simulink model "RCAM_PID_takeoff_lamding_20261013_step02"  (R2024b)
settings: Solver=VariableStepAuto  StartTime=0.0  StopTime=4200  MaxStep=0.01  RelTol=1e-3
undefined symbols (not defined in the file or in its folder): RCAM_dynamics_fcn20261013_step02_brake, RCAM_monitor_20261013_step02
libraries: simulink x28, slpidlib x9, simulink_extras x2
(part 1 of 2)
settings Model: Creator=rukky  LastModifiedBy=rukky
settings SolverCC: ZeroCrossAlgorithm=Adaptive
settings DebuggingCC: MaskedZcDiagnostic=none  IgnoredZcDiagnostic=none

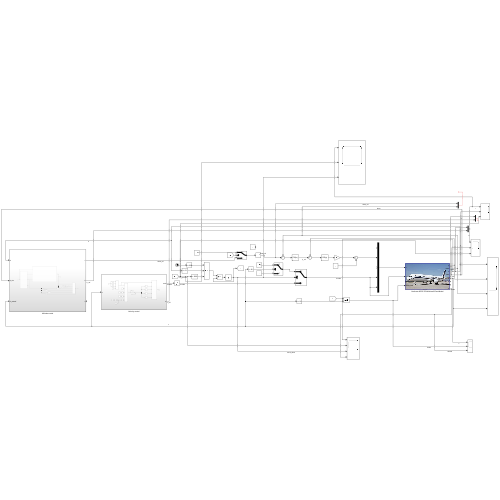
[thumbnail: Simulink's stored preview of the top-level diagram]
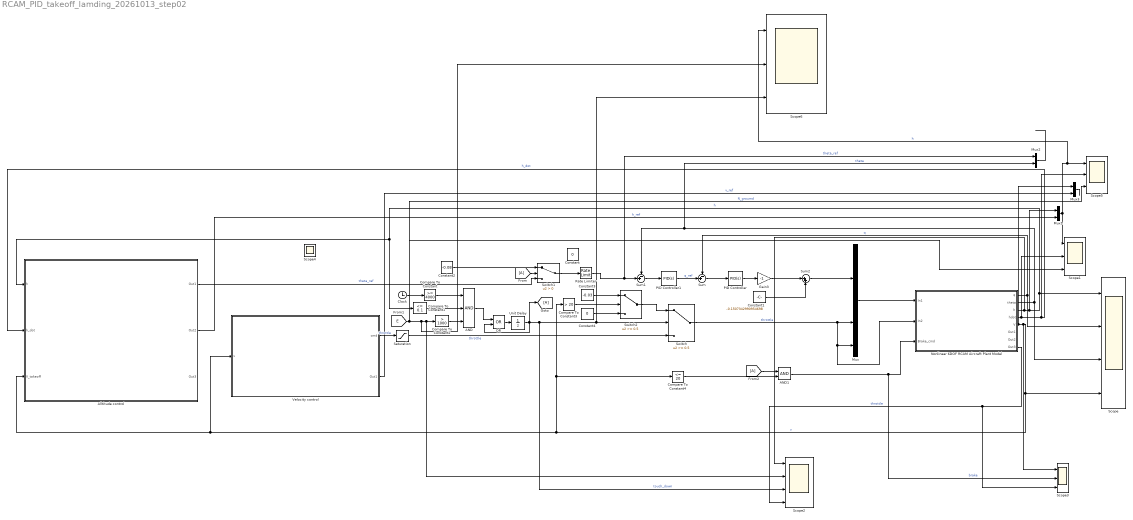
== system RCAM_PID_takeoff_lamding_20261013_step02 ==
  AND : Logic  Inputs=3  AllPortsSameDT=off  OutDataTypeStr=boolean
  AND1 : Logic  AllPortsSameDT=off  OutDataTypeStr=boolean
  Alltitude control : Subsystem
  Clock : Clock
  Compare To Constant : simulink/Logic and Bit Operations/Compare To Constant  relop=>=  const=4000  OutDataTypeStr=boolean
  Compare To Constant1 : simulink/Logic and Bit Operations/Compare To Constant  relop=<=  const=0.1  OutDataTypeStr=boolean
  Compare To Constant2 : simulink/Logic and Bit Operations/Compare To Constant  relop=>  const=1000  OutDataTypeStr=boolean
  Compare To Constant3 : simulink/Logic and Bit Operations/Compare To Constant  relop=>  const=20  OutDataTypeStr=boolean
  Compare To Constant4 : simulink/Logic and Bit Operations/Compare To Constant  relop=<=  const=20  OutDataTypeStr=boolean
  Constant : Constant  Value=0
  Constant1 : Constant  Value=-0.1507342990954698
  Constant2 : Constant  Value=-0.08
  Constant3 : Constant  Value=-0.03
  Constant4 : Constant  Value=0
  From : From
  From2 : From
  Gain3 : Gain  Gain=-1
  Goto : Goto
  Mux : Mux  Inputs=5
  Mux1 : Mux  Inputs=2
  Mux2 : Mux  Inputs=2
  Mux3 : Mux  Inputs=2
  Nonlinear 6DOF RCAM Aircraft Plant Model : Subsystem
      mask Display: image('$imagefile'); % Use "Edit Image" on toolstrip to change.
  OR : Logic  Operator=OR  AllPortsSameDT=off  OutDataTypeStr=boolean
  PID Controller : slpidlib/PID Controller  Controller=PID  Form=Parallel  TimeDomain=Continuous-time  UseExternalTs=off  SampleTime=-1  IntegratorMethod=Forward Euler  FilterMethod=Forward Euler  ControllerParametersSource=internal  P=20  I=20  UseKiTs=off  D=0  UseExternalDerivativeSource=off  N=100  UseFilter=on  TunerSelectOption=Transfer Function Based (PID Tuner App)  InitialConditionSource=internal  InitialConditionForIntegrator=0  InitialConditionForFilter=0  DifferentiatorICPrevScaledInput=0  ExternalReset=none  TrackingMode=off  Kt=1  LimitOutput=off  SatLimitsSource=internal  UpperSaturationLimit=inf  LowerSaturationLimit=-inf  LinearizeAsGain=on  AntiWindupMode=none  Kb=1  LimitIntegrator=off  UpperIntegratorSaturationLimit=inf  LowerIntegratorSaturationLimit=-inf  POutMin=[]  POutMax=[]  IOutMin=[]  IOutMax=[]  DOutMin=[]  DOutMax=[]  NOutMin=[]  NOutMax=[]  SumOutMin=[]  SumOutMax=[]  SaturationOutMin=[]  SaturationOutMax=[]  PParamMin=[]  PParamMax=[]  IParamMin=[]  IParamMax=[]  DParamMin=[]  DParamMax=[]  NParamMin=[]  NParamMax=[]  KbParamMin=[]  KbParamMax=[]  KtParamMin=[]  KtParamMax=[]  KbOutMin=[]  KbOutMax=[]  KtOutMin=[]  KtOutMax=[]  IntegratorOutMin=[]  IntegratorOutMax=[]  FilterOutMin=[]  FilterOutMax=[]  SumI1OutMin=[]  SumI1OutMax=[]  SumI2OutMin=[]  SumI2OutMax=[]  SumI3OutMin=[]  SumI3OutMax=[]  SumI4OutMin=[]  SumI4OutMax=[]  SumDOutMin=[]  SumDOutMax=[]  DifferentiatorOutMin=[]  DifferentiatorOutMax=[]  FilterDiffOutCoefMin=[]  FilterDiffOutCoefMax=[]  ReciprocalOutMin=[]  ReciprocalOutMax=[]  SumDenOutMin=[]  SumDenOutMax=[]  SumNumOutMin=[]  SumNumOutMax=[]  DivideOutMin=[]  DivideOutMax=[]  UdiffTsProdOutMin=[]  UdiffTsProdOutMax=[]  NTsProdOutMin=[]  NTsProdOutMax=[]  UintegralTsProdOutMin=[]  UintegralTsProdOutMax=[]  UngainTsProdOutMin=[]  UngainTsProdOutMax=[]  ClampingZeroOutDataTypeStr=Inherit: Inherit via back propagation  ClampingZeroOutMin=[]  ClampingZeroOutMax=[]  FilterDenConstantOutDataTypeStr=Inherit: Inherit via back propagation  FilterDenConstantOutMin=[]  FilterDenConstantOutMax=[]  PCopyOutDataTypeStr=Inherit: Inherit via back propagation  PCopyOutMin=[]  PCopyOutMax=[]  NCopyOutDataTypeStr=Inherit: Inherit via back propagation  NCopyOutMin=[]  NCopyOutMax=[]  IntegratorContinuousStateAttributes=''  IntegratorStateMustResolveToSignalObject=off  IntegratorRTWStateStorageClass=Auto  FilterContinuousStateAttributes=''  FilterStateMustResolveToSignalObject=off  FilterRTWStateStorageClass=Auto  ParallelPVariant=InternalParameters  IdealPVariant=Disabled  IVariant=InternalParameters  DVariant=InternalParameters  IntegratorVariant=Continuous  SatVariant=Disabled  AWVariant=Passthrough  PCopyVariant=Disabled  TRVariant=Disabled  FdbkBlocksVariant=Forward  IdealPFdbkVariant=Disabled  SatFdbkVariant=Disabled  DerivativeFilterVariant=ContFilter  NVariant=InternalParameters  NCopyVariant=Disabled  FilterICVariant=InternalICsFilter  IntegratorICVariant=InternalICs  ExternalResetVariant=Disabled  TRSumVariant=Passthrough  SumFdbkVariant=Disabled  SumVariant=Sum_PID  TsampFilterVariant=InternalTs  TsampNgainVariant=Passthrough  TsampIntegralVariant=Disabled_SignalSpec  ExternalSaturationOutDataTypeStr=Inherit: Same as second input  DerivativeSourceVariant=ErrorSignal  PreIntVariant=InternalPreInt
  PID Controller1 : slpidlib/PID Controller  Controller=PID  Form=Parallel  TimeDomain=Continuous-time  UseExternalTs=off  SampleTime=-1  IntegratorMethod=Forward Euler  FilterMethod=Forward Euler  ControllerParametersSource=internal  P=1  I=0  UseKiTs=off  D=0  UseExternalDerivativeSource=off  N=100  UseFilter=on  TunerSelectOption=Transfer Function Based (PID Tuner App)  InitialConditionSource=internal  InitialConditionForIntegrator=0  InitialConditionForFilter=0  DifferentiatorICPrevScaledInput=0  ExternalReset=none  TrackingMode=off  Kt=1  LimitOutput=off  SatLimitsSource=internal  UpperSaturationLimit=inf  LowerSaturationLimit=-inf  LinearizeAsGain=on  AntiWindupMode=none  Kb=1  LimitIntegrator=off  UpperIntegratorSaturationLimit=inf  LowerIntegratorSaturationLimit=-inf  POutMin=[]  POutMax=[]  IOutMin=[]  IOutMax=[]  DOutMin=[]  DOutMax=[]  NOutMin=[]  NOutMax=[]  SumOutMin=[]  SumOutMax=[]  SaturationOutMin=[]  SaturationOutMax=[]  PParamMin=[]  PParamMax=[]  IParamMin=[]  IParamMax=[]  DParamMin=[]  DParamMax=[]  NParamMin=[]  NParamMax=[]  KbParamMin=[]  KbParamMax=[]  KtParamMin=[]  KtParamMax=[]  KbOutMin=[]  KbOutMax=[]  KtOutMin=[]  KtOutMax=[]  IntegratorOutMin=[]  IntegratorOutMax=[]  FilterOutMin=[]  FilterOutMax=[]  SumI1OutMin=[]  SumI1OutMax=[]  SumI2OutMin=[]  SumI2OutMax=[]  SumI3OutMin=[]  SumI3OutMax=[]  SumI4OutMin=[]  SumI4OutMax=[]  SumDOutMin=[]  SumDOutMax=[]  DifferentiatorOutMin=[]  DifferentiatorOutMax=[]  FilterDiffOutCoefMin=[]  FilterDiffOutCoefMax=[]  ReciprocalOutMin=[]  ReciprocalOutMax=[]  SumDenOutMin=[]  SumDenOutMax=[]  SumNumOutMin=[]  SumNumOutMax=[]  DivideOutMin=[]  DivideOutMax=[]  UdiffTsProdOutMin=[]  UdiffTsProdOutMax=[]  NTsProdOutMin=[]  NTsProdOutMax=[]  UintegralTsProdOutMin=[]  UintegralTsProdOutMax=[]  UngainTsProdOutMin=[]  UngainTsProdOutMax=[]  ClampingZeroOutDataTypeStr=Inherit: Inherit via back propagation  ClampingZeroOutMin=[]  ClampingZeroOutMax=[]  FilterDenConstantOutDataTypeStr=Inherit: Inherit via back propagation  FilterDenConstantOutMin=[]  FilterDenConstantOutMax=[]  PCopyOutDataTypeStr=Inherit: Inherit via back propagation  PCopyOutMin=[]  PCopyOutMax=[]  NCopyOutDataTypeStr=Inherit: Inherit via back propagation  NCopyOutMin=[]  NCopyOutMax=[]  IntegratorContinuousStateAttributes=''  IntegratorStateMustResolveToSignalObject=off  IntegratorRTWStateStorageClass=Auto  FilterContinuousStateAttributes=''  FilterStateMustResolveToSignalObject=off  FilterRTWStateStorageClass=Auto  ParallelPVariant=InternalParameters  IdealPVariant=Disabled  IVariant=InternalParameters  DVariant=InternalParameters  IntegratorVariant=Continuous  SatVariant=Disabled  AWVariant=Passthrough  PCopyVariant=Disabled  TRVariant=Disabled  FdbkBlocksVariant=Forward  IdealPFdbkVariant=Disabled  SatFdbkVariant=Disabled  DerivativeFilterVariant=ContFilter  NVariant=InternalParameters  NCopyVariant=Disabled  FilterICVariant=InternalICsFilter  IntegratorICVariant=InternalICs  ExternalResetVariant=Disabled  TRSumVariant=Passthrough  SumFdbkVariant=Disabled  SumVariant=Sum_PID  TsampFilterVariant=InternalTs  TsampNgainVariant=Passthrough  TsampIntegralVariant=Disabled_SignalSpec  ExternalSaturationOutDataTypeStr=Inherit: Same as second input  DerivativeSourceVariant=ErrorSignal  PreIntVariant=InternalPreInt
  Rate Limiter : RateLimiter  RisingSlewLimit=2*pi/180  FallingSlewLimit=-2*pi/180  SampleTimeMode=inherited
  Saturation : Saturate  UpperLimit=1  LowerLimit=0
  Scope : Scope  NumInputPorts=4
  Scope{1,3,5..6} (4 alike) : Scope  NumInputPorts=3
  Scope2 : Scope  NumInputPorts=4
  Sum : Sum  Inputs=-+|
  Sum1 : Sum  Inputs=-+|
  Sum2 : Sum  Inputs=|++
  Switch : Switch  Threshold=0.5  SaturateOnIntegerOverflow=off  InputSameDT=off
  Switch1 : Switch  Criteria=u2 > Threshold  SaturateOnIntegerOverflow=off  InputSameDT=off
  Switch2 : Switch  Threshold=0.5  SaturateOnIntegerOverflow=off  InputSameDT=off
  Unit Delay : UnitDelay  SampleTime=0.01  HasFrameUpgradeWarning=on
  Velocity control : Subsystem
  Scope4 : Scope
  wires:
  PID Controller1/1 -> Sum/2  "q_ref"
  Sum1/1 -> PID Controller1/1
  PID Controller/1 -> Gain3/1
  Gain3/1 -> Sum2/1
  Sum/1 -> PID Controller/1
  Mux/1 -> Nonlinear 6DOF RCAM Aircraft Plant Model/1(In1)
  Nonlinear 6DOF RCAM Aircraft Plant Model/1(q) -> Scope/2, Sum/1  "q"
  Nonlinear 6DOF RCAM Aircraft Plant Model/2(theta) -> Mux2/2, Sum1/1, Scope/3  "theta"
  Nonlinear 6DOF RCAM Aircraft Plant Model/3(h) -> Scope2/1, Mux1/1, Scope/1, Alltitude control/1(h), Compare To Constant1/1  "h"
  Rate Limiter/1 -> Mux2/1, Sum1/2  "theta_ref"
  Switch/1 -> Nonlinear 6DOF RCAM Aircraft Plant Model/2(In2), Mux/5, Mux/4  "throttle"
  Nonlinear 6DOF RCAM Aircraft Plant Model/5(V) -> Mux3/1, Scope3/1, Scope/4, Alltitude control/3(V_takeoff), Velocity control/1(v), Compare To Constant3/1, Compare To Constant4/1  "v"
  Nonlinear 6DOF RCAM Aircraft Plant Model/4(hdot) -> Scope1/2, Scope5/2, Alltitude control/2(h_dot)  "h_dot"
  Sum2/1 -> Mux/2
  Constant1/1 -> Sum2/2
  Alltitude control/1(Out1) -> Switch1/3  "theta_ref"
  AND/1 -> OR/1
  OR/1 -> Unit Delay/1
  Unit Delay/1 -> Scope2/3, Scope6/3, Switch/2, Goto/1, OR/2  "touch_down"
  Velocity control/1(cmd) -> Saturation/1  "throttle"
  Saturation/1 -> Switch/3  "throttle"
  Clock/1 -> Compare To Constant/1
  Compare To Constant/1 -> AND/1
  Compare To Constant1/1 -> AND/2
  [E] -> Scope1/3, Scope6/2, Scope2/2, Compare To Constant2/1, Scope5/3  "N_groumd"
  Compare To Constant2/1 -> AND/3
  Switch1/1 -> Rate Limiter/1
  Constant2/1 -> Switch1/1
  Compare To Constant3/1 -> Switch2/2
  Constant3/1 -> Switch2/1
  Constant4/1 -> Switch2/3
  Switch2/1 -> Switch/1
  Compare To Constant4/1 -> AND1/2
  AND1/1 -> Scope3/2, Nonlinear 6DOF RCAM Aircraft Plant Model/3(Brake_cmd)  "brake"
  From/1 -> Switch1/2
  From2/1 -> AND1/1
  Alltitude control/2(Out2) -> Mux1/2  "h_ref"
  Mux1/1 -> Scope1/1, Scope6/1, Scope5/1  "h"
  Nonlinear 6DOF RCAM Aircraft Plant Model/8(Out3) -> Scope3/3, Scope2/4  "throttle"
  Mux2/1 -> ?
  Mux3/1 -> ?
  Velocity control/2(Out1) -> Mux3/2  "v_ref"

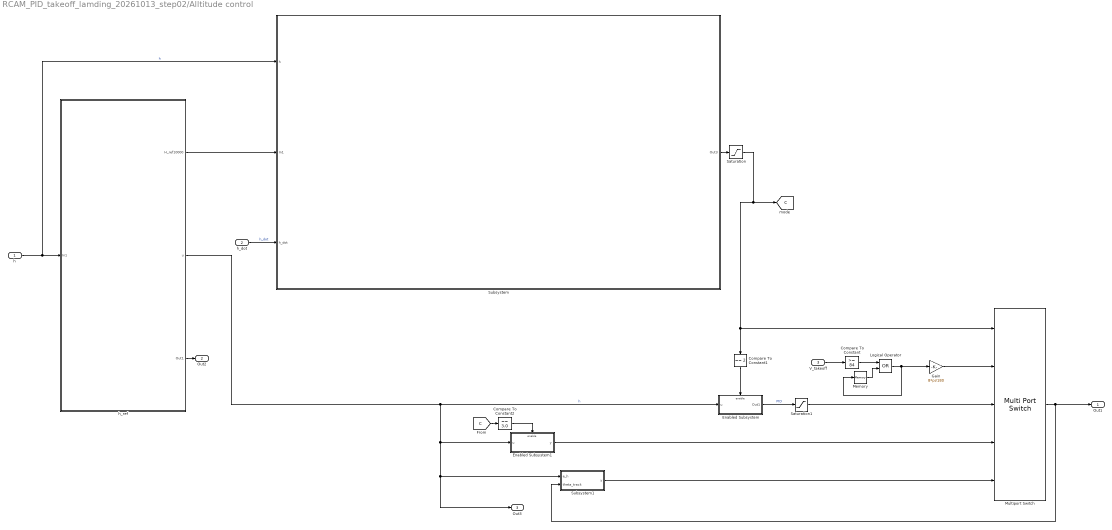
== system RCAM_PID_takeoff_lamding_20261013_step02/Alltitude control ==
  h : Inport
  h_dot : Inport  Port=2
  V_takeoff : Inport  Port=3
  Compare To Constant : simulink/Logic and Bit Operations/Compare To Constant  relop=>=  const=84  OutDataTypeStr=boolean
  Compare To Constant1 : simulink/Logic and Bit Operations/Compare To Constant  relop===  const=2  OutDataTypeStr=boolean
  Compare To Constant2 : simulink/Logic and Bit Operations/Compare To Constant  relop===  const=3.0  OutDataTypeStr=boolean
  Enabled Subsystem : Subsystem  TreatAsAtomicUnit=on
  Enabled Subsystem1 : Subsystem  TreatAsAtomicUnit=on
  Gain : Gain  Gain=8*pi/180
  Logical Operator : Logic  Operator=OR  AllPortsSameDT=off  OutDataTypeStr=boolean
  Memory : Memory
  Multiport Switch : MultiPortSwitch  Inputs=4  SaturateOnIntegerOverflow=off  InputSameDT=off
  Saturation : Saturate  UpperLimit=4  LowerLimit=1
  Saturation1 : Saturate  UpperLimit=0.175  LowerLimit=-0.175
  Subsystem : Subsystem
  Subsystem1 : Subsystem
  h_ref : Subsystem
  Out1 : Outport
  Out2 : Outport  Port=2
  Out3 : Outport  Port=3
  tag scope: C=global
  wires:
  h/1 -> Subsystem/1(h), h_ref/1(In1)  "h"
  h_ref/1(H_ref10000) -> Subsystem/2(In1)
  h_dot/1 -> Subsystem/3(h_dot)  "h_dot"
  Saturation/1 -> Compare To Constant1/1, Multiport Switch/1, [C]
  Saturation1/1 -> Multiport Switch/3
  Enabled Subsystem1/1(y) -> Multiport Switch/4
  h_ref/2(u) -> Out3/1, Subsystem1/1(e_h), Enabled Subsystem1/1(u), Enabled Subsystem/1(u)  "h"
  Enabled Subsystem/1(Out1) -> Saturation1/1  "PID"
  Gain/1 -> Multiport Switch/2
  V_takeoff/1 -> Compare To Constant/1
  Multiport Switch/1 -> Out1/1, Subsystem1/2(theta_track)
  Compare To Constant/1 -> Logical Operator/1
  Memory/1 -> Logical Operator/2
  Logical Operator/1 -> Memory/1, Gain/1
  h_ref/3(Out1) -> Out2/1
  Subsystem/1(Out3) -> Saturation/1
  Compare To Constant1/1 -> Enabled Subsystem/Enable
  Compare To Constant2/1 -> Enabled Subsystem1/Enable
  Subsystem1/1(y) -> Multiport Switch/5
  [C] -> Compare To Constant2/1

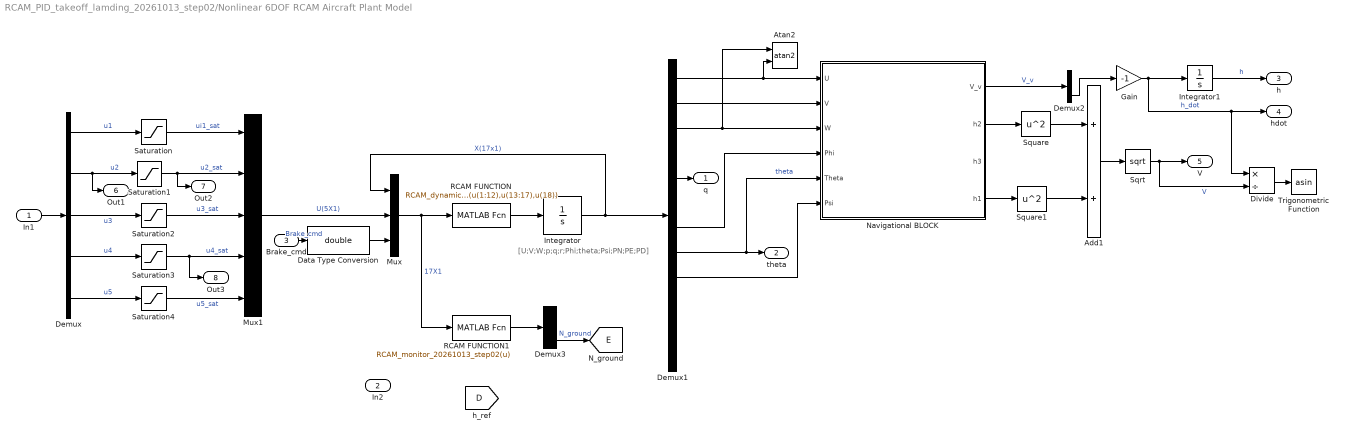
== system RCAM_PID_takeoff_lamding_20261013_step02/Nonlinear 6DOF RCAM Aircraft Plant Model ==
  note: [U;V;W;p;q;r;Phi;theta;Psi;PN;PE;PD]
  In1 : Inport
  In2 : Inport  Port=2
  Brake_cmd : Inport  Port=3
  Add1 : Sum
  Atan2 : Trigonometry  Operator=atan2
  Data Type Conversion : DataTypeConversion  OutDataTypeStr=double  SaturateOnIntegerOverflow=off  RndMeth=Floor
  Demux : Demux  Outputs=5
  Demux1 : Demux  Outputs=12
  Demux2 : Demux  Outputs=3
  Demux3 : Demux  Outputs=3
  Divide : Product  Inputs=*/
  Gain : Gain  Gain=-1
  Integrator : Integrator  InitialCondition=[77.0814;0;0;0;0;0;0;0;0;0;0;0]
  Integrator1 : Integrator
  Mux : Mux  Inputs=3
  Mux1 : Mux  Inputs=5
  Navigational BLOCK : Subsystem
  RCAM FUNCTION : MATLABFcn  MATLABFcn=RCAM_dynamics_fcn20261013_step02_brake(u(1:12),u(13:17),u(18))
  RCAM FUNCTION1 : MATLABFcn  MATLABFcn=RCAM_monitor_20261013_step02(u)  OutputDimensions=3
  Saturation : Saturate  UpperLimit=25*(pi/180)  LowerLimit=-15*(pi/180)
  Saturation1 : Saturate  UpperLimit=10*(pi/180)  LowerLimit=-25*(pi/180)
  Saturation2 : Saturate  UpperLimit=30*(pi/180)  LowerLimit=-30*(pi/180)
  Saturation3 : Saturate  UpperLimit=1  LowerLimit=-0.03
  Saturation4 : Saturate  UpperLimit=1  LowerLimit=-0.03
  Sqrt : Sqrt
  Square : Math  Operator=square
  Square1 : Math  Operator=square
  Trigonometric Function : Trigonometry  Operator=asin
  q : Outport
  theta : Outport  Port=2
  h : Outport  Port=3
  hdot : Outport  Port=4
  V : Outport  Port=5
  Out1 : Outport  Port=6
  Out2 : Outport  Port=7
  Out3 : Outport  Port=8
  tag scope: E=global
  wires:
  Integrator/1 -> Mux/1, Demux1/1  "X(17x1)"
  Demux/1 -> Saturation/1  "u1"
  Saturation/1 -> Mux1/1  "ui1_sat"
  Demux/2 -> Saturation1/1, Out1/1  "u2"
  Demux/3 -> Saturation2/1  "u3"
  Demux/4 -> Saturation3/1  "u4"
  Demux/5 -> Saturation4/1  "u5"
  Saturation1/1 -> Mux1/2, Out2/1  "u2_sat"
  Saturation2/1 -> Mux1/3  "u3_sat"
  Saturation3/1 -> Mux1/4, Out3/1  "u4_sat"
  Saturation4/1 -> Mux1/5  "u5_sat"
  RCAM FUNCTION/1 -> Integrator/1
  Mux1/1 -> Mux/2  "U(5X1)"
  In1/1 -> Demux/1
  Demux1/3 -> Atan2/1, Navigational BLOCK/3(W)
  Demux1/5 -> q/1
  Demux1/8 -> theta/1, Navigational BLOCK/5(Theta)  "theta"
  Demux1/1 -> Atan2/2, Navigational BLOCK/1(U)
  Demux1/2 -> Navigational BLOCK/2(V)
  Demux1/7 -> Navigational BLOCK/4(Phi)
  Demux1/9 -> Navigational BLOCK/6(Psi)
  Demux2/3 -> Gain/1
  Navigational BLOCK/1(V_v) -> Demux2/1  "V_v"
  Integrator1/1 -> h/1  "h"
  Navigational BLOCK/2(h2) -> Square/1
  Square/1 -> Add1/1
  Add1/1 -> Sqrt/1
  Square1/1 -> Add1/2
  Navigational BLOCK/4(h1) -> Square1/1
  Mux/1 -> RCAM FUNCTION1/1, RCAM FUNCTION/1  "17X1"
  RCAM FUNCTION1/1 -> Demux3/1
  Demux3/3 -> [E]  "N_ground"
  Sqrt/1 -> Divide/2, V/1  "V"
  Gain/1 -> hdot/1, Divide/1, Integrator1/1  "h_dot"
  Divide/1 -> Trigonometric Function/1
  Brake_cmd/1 -> Data Type Conversion/1  "Brake_cmd"
  Data Type Conversion/1 -> Mux/3

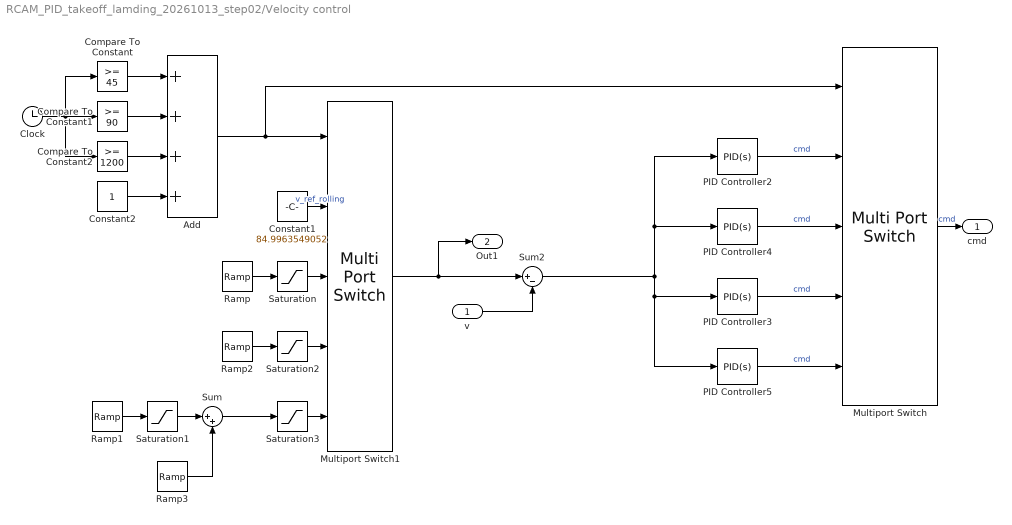
== system RCAM_PID_takeoff_lamding_20261013_step02/Velocity control ==
  v : Inport
  Add : Sum  Inputs=++++
  Clock : Clock
  Compare To Constant : simulink/Logic and Bit Operations/Compare To Constant  relop=>=  const=45  OutDataTypeStr=boolean
  Compare To Constant1 : simulink/Logic and Bit Operations/Compare To Constant  relop=>=  const=90  OutDataTypeStr=boolean
  Compare To Constant2 : simulink/Logic and Bit Operations/Compare To Constant  relop=>=  const=1200  OutDataTypeStr=boolean
  Constant1 : Constant  Value=84.9963549052
  Constant2 : Constant
  Multiport Switch : MultiPortSwitch  Inputs=4  SaturateOnIntegerOverflow=off  InputSameDT=off
  Multiport Switch1 : MultiPortSwitch  Inputs=4  SaturateOnIntegerOverflow=off  InputSameDT=off
  PID Controller2 : slpidlib/PID Controller  Controller=PID  Form=Parallel  TimeDomain=Continuous-time  UseExternalTs=off  SampleTime=-1  IntegratorMethod=Forward Euler  FilterMethod=Forward Euler  ControllerParametersSource=internal  P=16e-1  I=1e-3  UseKiTs=off  D=0  UseExternalDerivativeSource=off  N=100  UseFilter=on  TunerSelectOption=Transfer Function Based (PID Tuner App)  InitialConditionSource=internal  InitialConditionForIntegrator=0  InitialConditionForFilter=0  DifferentiatorICPrevScaledInput=0  ExternalReset=none  TrackingMode=off  Kt=1  LimitOutput=off  SatLimitsSource=internal  UpperSaturationLimit=inf  LowerSaturationLimit=-inf  LinearizeAsGain=on  AntiWindupMode=none  Kb=1  LimitIntegrator=off  UpperIntegratorSaturationLimit=inf  LowerIntegratorSaturationLimit=-inf  POutMin=[]  POutMax=[]  IOutMin=[]  IOutMax=[]  DOutMin=[]  DOutMax=[]  NOutMin=[]  NOutMax=[]  SumOutMin=[]  SumOutMax=[]  SaturationOutMin=[]  SaturationOutMax=[]  PParamMin=[]  PParamMax=[]  IParamMin=[]  IParamMax=[]  DParamMin=[]  DParamMax=[]  NParamMin=[]  NParamMax=[]  KbParamMin=[]  KbParamMax=[]  KtParamMin=[]  KtParamMax=[]  KbOutMin=[]  KbOutMax=[]  KtOutMin=[]  KtOutMax=[]  IntegratorOutMin=[]  IntegratorOutMax=[]  FilterOutMin=[]  FilterOutMax=[]  SumI1OutMin=[]  SumI1OutMax=[]  SumI2OutMin=[]  SumI2OutMax=[]  SumI3OutMin=[]  SumI3OutMax=[]  SumI4OutMin=[]  SumI4OutMax=[]  SumDOutMin=[]  SumDOutMax=[]  DifferentiatorOutMin=[]  DifferentiatorOutMax=[]  FilterDiffOutCoefMin=[]  FilterDiffOutCoefMax=[]  ReciprocalOutMin=[]  ReciprocalOutMax=[]  SumDenOutMin=[]  SumDenOutMax=[]  SumNumOutMin=[]  SumNumOutMax=[]  DivideOutMin=[]  DivideOutMax=[]  UdiffTsProdOutMin=[]  UdiffTsProdOutMax=[]  NTsProdOutMin=[]  NTsProdOutMax=[]  UintegralTsProdOutMin=[]  UintegralTsProdOutMax=[]  UngainTsProdOutMin=[]  UngainTsProdOutMax=[]  ClampingZeroOutDataTypeStr=Inherit: Inherit via back propagation  ClampingZeroOutMin=[]  ClampingZeroOutMax=[]  FilterDenConstantOutDataTypeStr=Inherit: Inherit via back propagation  FilterDenConstantOutMin=[]  FilterDenConstantOutMax=[]  PCopyOutDataTypeStr=Inherit: Inherit via back propagation  PCopyOutMin=[]  PCopyOutMax=[]  NCopyOutDataTypeStr=Inherit: Inherit via back propagation  NCopyOutMin=[]  NCopyOutMax=[]  IntegratorContinuousStateAttributes=''  IntegratorStateMustResolveToSignalObject=off  IntegratorRTWStateStorageClass=Auto  FilterContinuousStateAttributes=''  FilterStateMustResolveToSignalObject=off  FilterRTWStateStorageClass=Auto  ParallelPVariant=InternalParameters  IdealPVariant=Disabled  IVariant=InternalParameters  DVariant=InternalParameters  IntegratorVariant=Continuous  SatVariant=Disabled  AWVariant=Passthrough  PCopyVariant=Disabled  TRVariant=Disabled  FdbkBlocksVariant=Forward  IdealPFdbkVariant=Disabled  SatFdbkVariant=Disabled  DerivativeFilterVariant=ContFilter  NVariant=InternalParameters  NCopyVariant=Disabled  FilterICVariant=InternalICsFilter  IntegratorICVariant=InternalICs  ExternalResetVariant=Disabled  TRSumVariant=Passthrough  SumFdbkVariant=Disabled  SumVariant=Sum_PID  TsampFilterVariant=InternalTs  TsampNgainVariant=Passthrough  TsampIntegralVariant=Disabled_SignalSpec  ExternalSaturationOutDataTypeStr=Inherit: Same as second input  DerivativeSourceVariant=ErrorSignal  PreIntVariant=InternalPreInt
  PID Controller3 : slpidlib/PID Controller  Controller=PID  Form=Parallel  TimeDomain=Continuous-time  UseExternalTs=off  SampleTime=-1  IntegratorMethod=Forward Euler  FilterMethod=Forward Euler  ControllerParametersSource=internal  P=1  I=0  UseKiTs=off  D=0  UseExternalDerivativeSource=off  N=100  UseFilter=on  TunerSelectOption=Transfer Function Based (PID Tuner App)  InitialConditionSource=internal  InitialConditionForIntegrator=0  InitialConditionForFilter=0  DifferentiatorICPrevScaledInput=0  ExternalReset=none  TrackingMode=off  Kt=1  LimitOutput=off  SatLimitsSource=internal  UpperSaturationLimit=inf  LowerSaturationLimit=-inf  LinearizeAsGain=on  AntiWindupMode=none  Kb=1  LimitIntegrator=off  UpperIntegratorSaturationLimit=inf  LowerIntegratorSaturationLimit=-inf  POutMin=[]  POutMax=[]  IOutMin=[]  IOutMax=[]  DOutMin=[]  DOutMax=[]  NOutMin=[]  NOutMax=[]  SumOutMin=[]  SumOutMax=[]  SaturationOutMin=[]  SaturationOutMax=[]  PParamMin=[]  PParamMax=[]  IParamMin=[]  IParamMax=[]  DParamMin=[]  DParamMax=[]  NParamMin=[]  NParamMax=[]  KbParamMin=[]  KbParamMax=[]  KtParamMin=[]  KtParamMax=[]  KbOutMin=[]  KbOutMax=[]  KtOutMin=[]  KtOutMax=[]  IntegratorOutMin=[]  IntegratorOutMax=[]  FilterOutMin=[]  FilterOutMax=[]  SumI1OutMin=[]  SumI1OutMax=[]  SumI2OutMin=[]  SumI2OutMax=[]  SumI3OutMin=[]  SumI3OutMax=[]  SumI4OutMin=[]  SumI4OutMax=[]  SumDOutMin=[]  SumDOutMax=[]  DifferentiatorOutMin=[]  DifferentiatorOutMax=[]  FilterDiffOutCoefMin=[]  FilterDiffOutCoefMax=[]  ReciprocalOutMin=[]  ReciprocalOutMax=[]  SumDenOutMin=[]  SumDenOutMax=[]  SumNumOutMin=[]  SumNumOutMax=[]  DivideOutMin=[]  DivideOutMax=[]  UdiffTsProdOutMin=[]  UdiffTsProdOutMax=[]  NTsProdOutMin=[]  NTsProdOutMax=[]  UintegralTsProdOutMin=[]  UintegralTsProdOutMax=[]  UngainTsProdOutMin=[]  UngainTsProdOutMax=[]  ClampingZeroOutDataTypeStr=Inherit: Inherit via back propagation  ClampingZeroOutMin=[]  ClampingZeroOutMax=[]  FilterDenConstantOutDataTypeStr=Inherit: Inherit via back propagation  FilterDenConstantOutMin=[]  FilterDenConstantOutMax=[]  PCopyOutDataTypeStr=Inherit: Inherit via back propagation  PCopyOutMin=[]  PCopyOutMax=[]  NCopyOutDataTypeStr=Inherit: Inherit via back propagation  NCopyOutMin=[]  NCopyOutMax=[]  IntegratorContinuousStateAttributes=''  IntegratorStateMustResolveToSignalObject=off  IntegratorRTWStateStorageClass=Auto  FilterContinuousStateAttributes=''  FilterStateMustResolveToSignalObject=off  FilterRTWStateStorageClass=Auto  ParallelPVariant=InternalParameters  IdealPVariant=Disabled  IVariant=InternalParameters  DVariant=InternalParameters  IntegratorVariant=Continuous  SatVariant=Disabled  AWVariant=Passthrough  PCopyVariant=Disabled  TRVariant=Disabled  FdbkBlocksVariant=Forward  IdealPFdbkVariant=Disabled  SatFdbkVariant=Disabled  DerivativeFilterVariant=ContFilter  NVariant=InternalParameters  NCopyVariant=Disabled  FilterICVariant=InternalICsFilter  IntegratorICVariant=InternalICs  ExternalResetVariant=Disabled  TRSumVariant=Passthrough  SumFdbkVariant=Disabled  SumVariant=Sum_PID  TsampFilterVariant=InternalTs  TsampNgainVariant=Passthrough  TsampIntegralVariant=Disabled_SignalSpec  ExternalSaturationOutDataTypeStr=Inherit: Same as second input  DerivativeSourceVariant=ErrorSignal  PreIntVariant=InternalPreInt
  PID Controller4 : slpidlib/PID Controller  Controller=PID  Form=Parallel  TimeDomain=Continuous-time  UseExternalTs=off  SampleTime=-1  IntegratorMethod=Forward Euler  FilterMethod=Forward Euler  ControllerParametersSource=internal  P=1  I=0  UseKiTs=off  D=0  UseExternalDerivativeSource=off  N=100  UseFilter=on  TunerSelectOption=Transfer Function Based (PID Tuner App)  InitialConditionSource=internal  InitialConditionForIntegrator=1  InitialConditionForFilter=0  DifferentiatorICPrevScaledInput=0  ExternalReset=none  TrackingMode=off  Kt=1  LimitOutput=off  SatLimitsSource=internal  UpperSaturationLimit=inf  LowerSaturationLimit=-inf  LinearizeAsGain=on  AntiWindupMode=none  Kb=1  LimitIntegrator=off  UpperIntegratorSaturationLimit=inf  LowerIntegratorSaturationLimit=-inf  POutMin=[]  POutMax=[]  IOutMin=[]  IOutMax=[]  DOutMin=[]  DOutMax=[]  NOutMin=[]  NOutMax=[]  SumOutMin=[]  SumOutMax=[]  SaturationOutMin=[]  SaturationOutMax=[]  PParamMin=[]  PParamMax=[]  IParamMin=[]  IParamMax=[]  DParamMin=[]  DParamMax=[]  NParamMin=[]  NParamMax=[]  KbParamMin=[]  KbParamMax=[]  KtParamMin=[]  KtParamMax=[]  KbOutMin=[]  KbOutMax=[]  KtOutMin=[]  KtOutMax=[]  IntegratorOutMin=[]  IntegratorOutMax=[]  FilterOutMin=[]  FilterOutMax=[]  SumI1OutMin=[]  SumI1OutMax=[]  SumI2OutMin=[]  SumI2OutMax=[]  SumI3OutMin=[]  SumI3OutMax=[]  SumI4OutMin=[]  SumI4OutMax=[]  SumDOutMin=[]  SumDOutMax=[]  DifferentiatorOutMin=[]  DifferentiatorOutMax=[]  FilterDiffOutCoefMin=[]  FilterDiffOutCoefMax=[]  ReciprocalOutMin=[]  ReciprocalOutMax=[]  SumDenOutMin=[]  SumDenOutMax=[]  SumNumOutMin=[]  SumNumOutMax=[]  DivideOutMin=[]  DivideOutMax=[]  UdiffTsProdOutMin=[]  UdiffTsProdOutMax=[]  NTsProdOutMin=[]  NTsProdOutMax=[]  UintegralTsProdOutMin=[]  UintegralTsProdOutMax=[]  UngainTsProdOutMin=[]  UngainTsProdOutMax=[]  ClampingZeroOutDataTypeStr=Inherit: Inherit via back propagation  ClampingZeroOutMin=[]  ClampingZeroOutMax=[]  FilterDenConstantOutDataTypeStr=Inherit: Inherit via back propagation  FilterDenConstantOutMin=[]  FilterDenConstantOutMax=[]  PCopyOutDataTypeStr=Inherit: Inherit via back propagation  PCopyOutMin=[]  PCopyOutMax=[]  NCopyOutDataTypeStr=Inherit: Inherit via back propagation  NCopyOutMin=[]  NCopyOutMax=[]  IntegratorContinuousStateAttributes=''  IntegratorStateMustResolveToSignalObject=off  IntegratorRTWStateStorageClass=Auto  FilterContinuousStateAttributes=''  FilterStateMustResolveToSignalObject=off  FilterRTWStateStorageClass=Auto  ParallelPVariant=InternalParameters  IdealPVariant=Disabled  IVariant=InternalParameters  DVariant=InternalParameters  IntegratorVariant=Continuous  SatVariant=Disabled  AWVariant=Passthrough  PCopyVariant=Disabled  TRVariant=Disabled  FdbkBlocksVariant=Forward  IdealPFdbkVariant=Disabled  SatFdbkVariant=Disabled  DerivativeFilterVariant=ContFilter  NVariant=InternalParameters  NCopyVariant=Disabled  FilterICVariant=InternalICsFilter  IntegratorICVariant=InternalICs  ExternalResetVariant=Disabled  TRSumVariant=Passthrough  SumFdbkVariant=Disabled  SumVariant=Sum_PID  TsampFilterVariant=InternalTs  TsampNgainVariant=Passthrough  TsampIntegralVariant=Disabled_SignalSpec  ExternalSaturationOutDataTypeStr=Inherit: Same as second input  DerivativeSourceVariant=ErrorSignal  PreIntVariant=InternalPreInt
  PID Controller5 : slpidlib/PID Controller  Controller=PID  Form=Parallel  TimeDomain=Continuous-time  UseExternalTs=off  SampleTime=-1  IntegratorMethod=Forward Euler  FilterMethod=Forward Euler  ControllerParametersSource=internal  P=1e-1  I=1e-3  UseKiTs=off  D=0  UseExternalDerivativeSource=off  N=100  UseFilter=on  TunerSelectOption=Transfer Function Based (PID Tuner App)  InitialConditionSource=internal  InitialConditionForIntegrator=0  InitialConditionForFilter=0  DifferentiatorICPrevScaledInput=0  ExternalReset=none  TrackingMode=off  Kt=1  LimitOutput=off  SatLimitsSource=internal  UpperSaturationLimit=inf  LowerSaturationLimit=-inf  LinearizeAsGain=on  AntiWindupMode=none  Kb=1  LimitIntegrator=off  UpperIntegratorSaturationLimit=inf  LowerIntegratorSaturationLimit=-inf  POutMin=[]  POutMax=[]  IOutMin=[]  IOutMax=[]  DOutMin=[]  DOutMax=[]  NOutMin=[]  NOutMax=[]  SumOutMin=[]  SumOutMax=[]  SaturationOutMin=[]  SaturationOutMax=[]  PParamMin=[]  PParamMax=[]  IParamMin=[]  IParamMax=[]  DParamMin=[]  DParamMax=[]  NParamMin=[]  NParamMax=[]  KbParamMin=[]  KbParamMax=[]  KtParamMin=[]  KtParamMax=[]  KbOutMin=[]  KbOutMax=[]  KtOutMin=[]  KtOutMax=[]  IntegratorOutMin=[]  IntegratorOutMax=[]  FilterOutMin=[]  FilterOutMax=[]  SumI1OutMin=[]  SumI1OutMax=[]  SumI2OutMin=[]  SumI2OutMax=[]  SumI3OutMin=[]  SumI3OutMax=[]  SumI4OutMin=[]  SumI4OutMax=[]  SumDOutMin=[]  SumDOutMax=[]  DifferentiatorOutMin=[]  DifferentiatorOutMax=[]  FilterDiffOutCoefMin=[]  FilterDiffOutCoefMax=[]  ReciprocalOutMin=[]  ReciprocalOutMax=[]  SumDenOutMin=[]  SumDenOutMax=[]  SumNumOutMin=[]  SumNumOutMax=[]  DivideOutMin=[]  DivideOutMax=[]  UdiffTsProdOutMin=[]  UdiffTsProdOutMax=[]  NTsProdOutMin=[]  NTsProdOutMax=[]  UintegralTsProdOutMin=[]  UintegralTsProdOutMax=[]  UngainTsProdOutMin=[]  UngainTsProdOutMax=[]  ClampingZeroOutDataTypeStr=Inherit: Inherit via back propagation  ClampingZeroOutMin=[]  ClampingZeroOutMax=[]  FilterDenConstantOutDataTypeStr=Inherit: Inherit via back propagation  FilterDenConstantOutMin=[]  FilterDenConstantOutMax=[]  PCopyOutDataTypeStr=Inherit: Inherit via back propagation  PCopyOutMin=[]  PCopyOutMax=[]  NCopyOutDataTypeStr=Inherit: Inherit via back propagation  NCopyOutMin=[]  NCopyOutMax=[]  IntegratorContinuousStateAttributes=''  IntegratorStateMustResolveToSignalObject=off  IntegratorRTWStateStorageClass=Auto  FilterContinuousStateAttributes=''  FilterStateMustResolveToSignalObject=off  FilterRTWStateStorageClass=Auto  ParallelPVariant=InternalParameters  IdealPVariant=Disabled  IVariant=InternalParameters  DVariant=InternalParameters  IntegratorVariant=Continuous  SatVariant=Disabled  AWVariant=Passthrough  PCopyVariant=Disabled  TRVariant=Disabled  FdbkBlocksVariant=Forward  IdealPFdbkVariant=Disabled  SatFdbkVariant=Disabled  DerivativeFilterVariant=ContFilter  NVariant=InternalParameters  NCopyVariant=Disabled  FilterICVariant=InternalICsFilter  IntegratorICVariant=InternalICs  ExternalResetVariant=Disabled  TRSumVariant=Passthrough  SumFdbkVariant=Disabled  SumVariant=Sum_PID  TsampFilterVariant=InternalTs  TsampNgainVariant=Passthrough  TsampIntegralVariant=Disabled_SignalSpec  ExternalSaturationOutDataTypeStr=Inherit: Same as second input  DerivativeSourceVariant=ErrorSignal  PreIntVariant=InternalPreInt
  Ramp : simulink/Sources/Ramp  slope=1  start=45  InitialOutput=90
  Ramp1 : simulink/Sources/Ramp  slope=-1  start=1200  InitialOutput=236
  Ramp2 : simulink/Sources/Ramp  slope=1  start=90  InitialOutput=120
  Ramp3 : simulink/Sources/Ramp  slope=-0.5  start=2700  InitialOutput=0
  Saturation : Saturate  UpperLimit=120  LowerLimit=90
  Saturation1 : Saturate  UpperLimit=236  LowerLimit=150
  Saturation2 : Saturate  UpperLimit=236  LowerLimit=120
  Saturation3 : Saturate  UpperLimit=236  LowerLimit=120
  Sum : Sum  Inputs=|++
  Sum2 : Sum  Inputs=|+-
  cmd : Outport
  Out1 : Outport  Port=2
  wires:
  Add/1 -> Multiport Switch/1, Multiport Switch1/1
  PID Controller2/1 -> Multiport Switch/2  "cmd"
  PID Controller4/1 -> Multiport Switch/3  "cmd"
  v/1 -> Sum2/2
  Multiport Switch1/1 -> Out1/1, Sum2/1
  PID Controller3/1 -> Multiport Switch/4  "cmd"
  PID Controller5/1 -> Multiport Switch/5  "cmd"
  Sum2/1 -> PID Controller3/1, PID Controller5/1, PID Controller4/1, PID Controller2/1
  Ramp2/1 -> Saturation2/1
  Constant2/1 -> Add/4
  Compare To Constant2/1 -> Add/3
  Compare To Constant1/1 -> Add/2
  Clock/1 -> Compare To Constant/1, Compare To Constant2/1, Compare To Constant1/1
  Ramp/1 -> Saturation/1
  Ramp1/1 -> Saturation1/1
  Saturation1/1 -> Sum/1
  Saturation/1 -> Multiport Switch1/3
  Saturation2/1 -> Multiport Switch1/4
  Compare To Constant/1 -> Add/1
  Constant1/1 -> Multiport Switch1/2  "v_ref_rolling"
  Multiport Switch/1 -> cmd/1  "cmd"
  Sum/1 -> Saturation3/1
  Ramp3/1 -> Sum/2
  Saturation3/1 -> Multiport Switch1/5

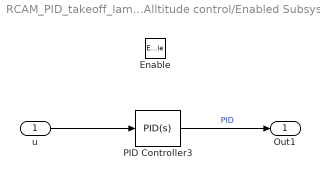
== system RCAM_PID_takeoff_lamding_20261013_step02/Alltitude control/Enabled Subsystem ==
  u : Inport
  Enable : EnablePort  StatesWhenEnabling=reset
  PID Controller3 : slpidlib/PID Controller  Controller=PID  Form=Parallel  TimeDomain=Continuous-time  UseExternalTs=off  SampleTime=-1  IntegratorMethod=Forward Euler  FilterMethod=Forward Euler  ControllerParametersSource=internal  P=4e-4  I=4e-6  UseKiTs=off  D=1e-2  UseExternalDerivativeSource=off  N=100  UseFilter=on  TunerSelectOption=Transfer Function Based (PID Tuner App)  InitialConditionSource=internal  InitialConditionForIntegrator=0  InitialConditionForFilter=0  DifferentiatorICPrevScaledInput=0  ExternalReset=none  TrackingMode=off  Kt=1  LimitOutput=off  SatLimitsSource=internal  UpperSaturationLimit=inf  LowerSaturationLimit=-inf  LinearizeAsGain=on  AntiWindupMode=none  Kb=1  LimitIntegrator=off  UpperIntegratorSaturationLimit=inf  LowerIntegratorSaturationLimit=-inf  POutMin=[]  POutMax=[]  IOutMin=[]  IOutMax=[]  DOutMin=[]  DOutMax=[]  NOutMin=[]  NOutMax=[]  SumOutMin=[]  SumOutMax=[]  SaturationOutMin=[]  SaturationOutMax=[]  PParamMin=[]  PParamMax=[]  IParamMin=[]  IParamMax=[]  DParamMin=[]  DParamMax=[]  NParamMin=[]  NParamMax=[]  KbParamMin=[]  KbParamMax=[]  KtParamMin=[]  KtParamMax=[]  KbOutMin=[]  KbOutMax=[]  KtOutMin=[]  KtOutMax=[]  IntegratorOutMin=[]  IntegratorOutMax=[]  FilterOutMin=[]  FilterOutMax=[]  SumI1OutMin=[]  SumI1OutMax=[]  SumI2OutMin=[]  SumI2OutMax=[]  SumI3OutMin=[]  SumI3OutMax=[]  SumI4OutMin=[]  SumI4OutMax=[]  SumDOutMin=[]  SumDOutMax=[]  DifferentiatorOutMin=[]  DifferentiatorOutMax=[]  FilterDiffOutCoefMin=[]  FilterDiffOutCoefMax=[]  ReciprocalOutMin=[]  ReciprocalOutMax=[]  SumDenOutMin=[]  SumDenOutMax=[]  SumNumOutMin=[]  SumNumOutMax=[]  DivideOutMin=[]  DivideOutMax=[]  UdiffTsProdOutMin=[]  UdiffTsProdOutMax=[]  NTsProdOutMin=[]  NTsProdOutMax=[]  UintegralTsProdOutMin=[]  UintegralTsProdOutMax=[]  UngainTsProdOutMin=[]  UngainTsProdOutMax=[]  ClampingZeroOutDataTypeStr=Inherit: Inherit via back propagation  ClampingZeroOutMin=[]  ClampingZeroOutMax=[]  FilterDenConstantOutDataTypeStr=Inherit: Inherit via back propagation  FilterDenConstantOutMin=[]  FilterDenConstantOutMax=[]  PCopyOutDataTypeStr=Inherit: Inherit via back propagation  PCopyOutMin=[]  PCopyOutMax=[]  NCopyOutDataTypeStr=Inherit: Inherit via back propagation  NCopyOutMin=[]  NCopyOutMax=[]  IntegratorContinuousStateAttributes=''  IntegratorStateMustResolveToSignalObject=off  IntegratorRTWStateStorageClass=Auto  FilterContinuousStateAttributes=''  FilterStateMustResolveToSignalObject=off  FilterRTWStateStorageClass=Auto  ParallelPVariant=InternalParameters  IdealPVariant=Disabled  IVariant=InternalParameters  DVariant=InternalParameters  IntegratorVariant=Continuous  SatVariant=Disabled  AWVariant=Passthrough  PCopyVariant=Disabled  TRVariant=Disabled  FdbkBlocksVariant=Forward  IdealPFdbkVariant=Disabled  SatFdbkVariant=Disabled  DerivativeFilterVariant=ContFilter  NVariant=InternalParameters  NCopyVariant=Disabled  FilterICVariant=InternalICsFilter  IntegratorICVariant=InternalICs  ExternalResetVariant=Disabled  TRSumVariant=Passthrough  SumFdbkVariant=Disabled  SumVariant=Sum_PID  TsampFilterVariant=InternalTs  TsampNgainVariant=Passthrough  TsampIntegralVariant=Disabled_SignalSpec  ExternalSaturationOutDataTypeStr=Inherit: Same as second input  DerivativeSourceVariant=ErrorSignal  PreIntVariant=InternalPreInt
  Out1 : Outport
  wires:
  u/1 -> PID Controller3/1
  PID Controller3/1 -> Out1/1  "PID"

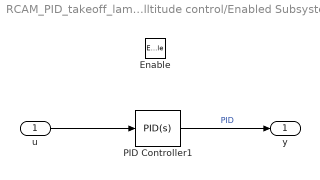
== system RCAM_PID_takeoff_lamding_20261013_step02/Alltitude control/Enabled Subsystem1 ==
  u : Inport
  Enable : EnablePort  StatesWhenEnabling=reset
  PID Controller1 : slpidlib/PID Controller  Controller=PID  Form=Parallel  TimeDomain=Continuous-time  UseExternalTs=off  SampleTime=-1  IntegratorMethod=Forward Euler  FilterMethod=Forward Euler  ControllerParametersSource=internal  P=4e-4  I=4e-6  UseKiTs=off  D=1e-3  UseExternalDerivativeSource=off  N=100  UseFilter=on  TunerSelectOption=Transfer Function Based (PID Tuner App)  InitialConditionSource=internal  InitialConditionForIntegrator=0  InitialConditionForFilter=0  DifferentiatorICPrevScaledInput=0  ExternalReset=none  TrackingMode=off  Kt=1  LimitOutput=off  SatLimitsSource=internal  UpperSaturationLimit=inf  LowerSaturationLimit=-inf  LinearizeAsGain=on  AntiWindupMode=none  Kb=1  LimitIntegrator=off  UpperIntegratorSaturationLimit=inf  LowerIntegratorSaturationLimit=-inf  POutMin=[]  POutMax=[]  IOutMin=[]  IOutMax=[]  DOutMin=[]  DOutMax=[]  NOutMin=[]  NOutMax=[]  SumOutMin=[]  SumOutMax=[]  SaturationOutMin=[]  SaturationOutMax=[]  PParamMin=[]  PParamMax=[]  IParamMin=[]  IParamMax=[]  DParamMin=[]  DParamMax=[]  NParamMin=[]  NParamMax=[]  KbParamMin=[]  KbParamMax=[]  KtParamMin=[]  KtParamMax=[]  KbOutMin=[]  KbOutMax=[]  KtOutMin=[]  KtOutMax=[]  IntegratorOutMin=[]  IntegratorOutMax=[]  FilterOutMin=[]  FilterOutMax=[]  SumI1OutMin=[]  SumI1OutMax=[]  SumI2OutMin=[]  SumI2OutMax=[]  SumI3OutMin=[]  SumI3OutMax=[]  SumI4OutMin=[]  SumI4OutMax=[]  SumDOutMin=[]  SumDOutMax=[]  DifferentiatorOutMin=[]  DifferentiatorOutMax=[]  FilterDiffOutCoefMin=[]  FilterDiffOutCoefMax=[]  ReciprocalOutMin=[]  ReciprocalOutMax=[]  SumDenOutMin=[]  SumDenOutMax=[]  SumNumOutMin=[]  SumNumOutMax=[]  DivideOutMin=[]  DivideOutMax=[]  UdiffTsProdOutMin=[]  UdiffTsProdOutMax=[]  NTsProdOutMin=[]  NTsProdOutMax=[]  UintegralTsProdOutMin=[]  UintegralTsProdOutMax=[]  UngainTsProdOutMin=[]  UngainTsProdOutMax=[]  ClampingZeroOutDataTypeStr=Inherit: Inherit via back propagation  ClampingZeroOutMin=[]  ClampingZeroOutMax=[]  FilterDenConstantOutDataTypeStr=Inherit: Inherit via back propagation  FilterDenConstantOutMin=[]  FilterDenConstantOutMax=[]  PCopyOutDataTypeStr=Inherit: Inherit via back propagation  PCopyOutMin=[]  PCopyOutMax=[]  NCopyOutDataTypeStr=Inherit: Inherit via back propagation  NCopyOutMin=[]  NCopyOutMax=[]  IntegratorContinuousStateAttributes=''  IntegratorStateMustResolveToSignalObject=off  IntegratorRTWStateStorageClass=Auto  FilterContinuousStateAttributes=''  FilterStateMustResolveToSignalObject=off  FilterRTWStateStorageClass=Auto  ParallelPVariant=InternalParameters  IdealPVariant=Disabled  IVariant=InternalParameters  DVariant=InternalParameters  IntegratorVariant=Continuous  SatVariant=Disabled  AWVariant=Passthrough  PCopyVariant=Disabled  TRVariant=Disabled  FdbkBlocksVariant=Forward  IdealPFdbkVariant=Disabled  SatFdbkVariant=Disabled  DerivativeFilterVariant=ContFilter  NVariant=InternalParameters  NCopyVariant=Disabled  FilterICVariant=InternalICsFilter  IntegratorICVariant=InternalICs  ExternalResetVariant=Disabled  TRSumVariant=Passthrough  SumFdbkVariant=Disabled  SumVariant=Sum_PID  TsampFilterVariant=InternalTs  TsampNgainVariant=Passthrough  TsampIntegralVariant=Disabled_SignalSpec  ExternalSaturationOutDataTypeStr=Inherit: Same as second input  DerivativeSourceVariant=ErrorSignal  PreIntVariant=InternalPreInt
  y : Outport
  wires:
  u/1 -> PID Controller1/1
  PID Controller1/1 -> y/1  "PID"

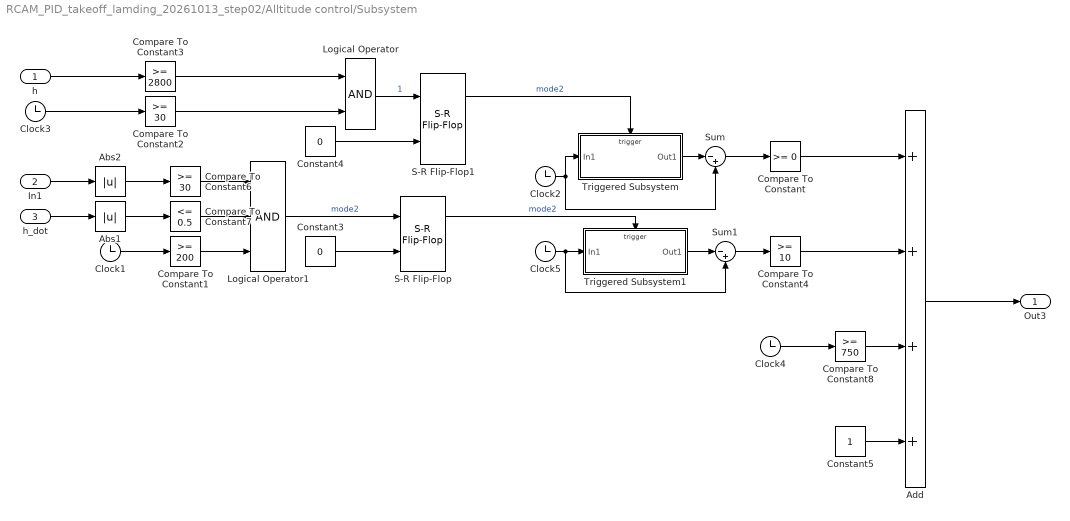
== system RCAM_PID_takeoff_lamding_20261013_step02/Alltitude control/Subsystem ==
  h : Inport
  In1 : Inport  Port=2
  h_dot : Inport  Port=3
  Abs1 : Abs  SaturateOnIntegerOverflow=off
  Abs2 : Abs  SaturateOnIntegerOverflow=off
  Add : Sum  Inputs=++++
  Clock{1..5} (5 alike) : Clock
  Compare To Constant : simulink/Logic and Bit Operations/Compare To Constant  relop=>=  const=0  OutDataTypeStr=boolean
  Compare To Constant1 : simulink/Logic and Bit Operations/Compare To Constant  relop=>=  const=200  OutDataTypeStr=boolean
  Compare To Constant2 : simulink/Logic and Bit Operations/Compare To Constant  relop=>=  const=30  OutDataTypeStr=boolean
  Compare To Constant3 : simulink/Logic and Bit Operations/Compare To Constant  relop=>=  const=2800  OutDataTypeStr=boolean
  Compare To Constant4 : simulink/Logic and Bit Operations/Compare To Constant  relop=>=  const=10  OutDataTypeStr=boolean
  Compare To Constant6 : simulink/Logic and Bit Operations/Compare To Constant  relop=>=  const=30  OutDataTypeStr=boolean
  Compare To Constant7 : simulink/Logic and Bit Operations/Compare To Constant  relop=<=  const=0.5  OutDataTypeStr=boolean
  Compare To Constant8 : simulink/Logic and Bit Operations/Compare To Constant  relop=>=  const=750  OutDataTypeStr=boolean
  Constant3 : Constant  Value=0  OutDataTypeStr=boolean
  Constant4 : Constant  Value=0  OutDataTypeStr=boolean
  Constant5 : Constant
  Logical Operator : Logic  AllPortsSameDT=off  OutDataTypeStr=boolean
  Logical Operator1 : Logic  Inputs=3  AllPortsSameDT=off  OutDataTypeStr=boolean
  S-R Flip-Flop : simulink_extras/Flip Flops/S-R Flip-Flop  initial_condition=0
  S-R Flip-Flop1 : simulink_extras/Flip Flops/S-R Flip-Flop  initial_condition=0
  Sum : Sum  Inputs=|-+
  Sum1 : Sum  Inputs=|-+
  Triggered Subsystem : Subsystem  TreatAsAtomicUnit=on
  Triggered Subsystem1 : Subsystem  TreatAsAtomicUnit=on
  Out3 : Outport
  wires:
  Constant3/1 -> S-R Flip-Flop/2
  S-R Flip-Flop1/1 -> Triggered Subsystem/Trigger  "mode2"
  S-R Flip-Flop/1 -> Triggered Subsystem1/Trigger  "mode2"
  Clock3/1 -> Compare To Constant2/1
  Sum1/1 -> Compare To Constant4/1
  Compare To Constant/1 -> Add/1
  Add/1 -> Out3/1
  Abs1/1 -> Compare To Constant7/1
  Clock4/1 -> Compare To Constant8/1
  h_dot/1 -> Abs1/1
  In1/1 -> Abs2/1
  Compare To Constant7/1 -> Logical Operator1/2
  Clock1/1 -> Compare To Constant1/1
  Logical Operator/1 -> S-R Flip-Flop1/1  "1"
  Compare To Constant8/1 -> Add/3
  Clock2/1 -> Sum/2, Triggered Subsystem/1(In1)
  Compare To Constant6/1 -> Logical Operator1/1
  Clock5/1 -> Sum1/2, Triggered Subsystem1/1(In1)
  Logical Operator1/1 -> S-R Flip-Flop/1  "mode2"
  Compare To Constant3/1 -> Logical Operator/1
  Constant4/1 -> S-R Flip-Flop1/2
  h/1 -> Compare To Constant3/1
  Triggered Subsystem1/1(Out1) -> Sum1/1
  Compare To Constant4/1 -> Add/2
  Sum/1 -> Compare To Constant/1
  Abs2/1 -> Compare To Constant6/1
  Compare To Constant1/1 -> Logical Operator1/3
  Triggered Subsystem/1(Out1) -> Sum/1
  Constant5/1 -> Add/4
  Compare To Constant2/1 -> Logical Operator/2

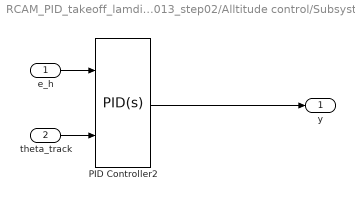
== system RCAM_PID_takeoff_lamding_20261013_step02/Alltitude control/Subsystem1 ==
  e_h : Inport
  theta_track : Inport  Port=2
  PID Controller2 : slpidlib/PID Controller  Controller=PID  Form=Parallel  TimeDomain=Continuous-time  UseExternalTs=off  SampleTime=-1  IntegratorMethod=Forward Euler  FilterMethod=Forward Euler  ControllerParametersSource=internal  P=4e-4  I=4e-6  UseKiTs=off  D=1e-3  UseExternalDerivativeSource=off  N=100  UseFilter=on  TunerSelectOption=Transfer Function Based (PID Tuner App)  InitialConditionSource=internal  InitialConditionForIntegrator=0  InitialConditionForFilter=0  DifferentiatorICPrevScaledInput=0  ExternalReset=none  TrackingMode=on  Kt=1  LimitOutput=off  SatLimitsSource=internal  UpperSaturationLimit=inf  LowerSaturationLimit=-inf  LinearizeAsGain=on  AntiWindupMode=none  Kb=1  LimitIntegrator=off  UpperIntegratorSaturationLimit=inf  LowerIntegratorSaturationLimit=-inf  POutMin=[]  POutMax=[]  IOutMin=[]  IOutMax=[]  DOutMin=[]  DOutMax=[]  NOutMin=[]  NOutMax=[]  SumOutMin=[]  SumOutMax=[]  SaturationOutMin=[]  SaturationOutMax=[]  PParamMin=[]  PParamMax=[]  IParamMin=[]  IParamMax=[]  DParamMin=[]  DParamMax=[]  NParamMin=[]  NParamMax=[]  KbParamMin=[]  KbParamMax=[]  KtParamMin=[]  KtParamMax=[]  KbOutMin=[]  KbOutMax=[]  KtOutMin=[]  KtOutMax=[]  IntegratorOutMin=[]  IntegratorOutMax=[]  FilterOutMin=[]  FilterOutMax=[]  SumI1OutMin=[]  SumI1OutMax=[]  SumI2OutMin=[]  SumI2OutMax=[]  SumI3OutMin=[]  SumI3OutMax=[]  SumI4OutMin=[]  SumI4OutMax=[]  SumDOutMin=[]  SumDOutMax=[]  DifferentiatorOutMin=[]  DifferentiatorOutMax=[]  FilterDiffOutCoefMin=[]  FilterDiffOutCoefMax=[]  ReciprocalOutMin=[]  ReciprocalOutMax=[]  SumDenOutMin=[]  SumDenOutMax=[]  SumNumOutMin=[]  SumNumOutMax=[]  DivideOutMin=[]  DivideOutMax=[]  UdiffTsProdOutMin=[]  UdiffTsProdOutMax=[]  NTsProdOutMin=[]  NTsProdOutMax=[]  UintegralTsProdOutMin=[]  UintegralTsProdOutMax=[]  UngainTsProdOutMin=[]  UngainTsProdOutMax=[]  ClampingZeroOutDataTypeStr=Inherit: Inherit via back propagation  ClampingZeroOutMin=[]  ClampingZeroOutMax=[]  FilterDenConstantOutDataTypeStr=Inherit: Inherit via back propagation  FilterDenConstantOutMin=[]  FilterDenConstantOutMax=[]  PCopyOutDataTypeStr=Inherit: Inherit via back propagation  PCopyOutMin=[]  PCopyOutMax=[]  NCopyOutDataTypeStr=Inherit: Inherit via back propagation  NCopyOutMin=[]  NCopyOutMax=[]  IntegratorContinuousStateAttributes=''  IntegratorStateMustResolveToSignalObject=off  IntegratorRTWStateStorageClass=Auto  FilterContinuousStateAttributes=''  FilterStateMustResolveToSignalObject=off  FilterRTWStateStorageClass=Auto  ParallelPVariant=InternalParameters  IdealPVariant=Disabled  IVariant=InternalParameters  DVariant=InternalParameters  IntegratorVariant=Continuous  SatVariant=Disabled  AWVariant=Passthrough  PCopyVariant=Disabled  TRVariant=Enabled  FdbkBlocksVariant=Forward  IdealPFdbkVariant=Disabled  SatFdbkVariant=Disabled  DerivativeFilterVariant=ContFilter  NVariant=InternalParameters  NCopyVariant=Disabled  FilterICVariant=InternalICsFilter  IntegratorICVariant=InternalICs  ExternalResetVariant=Disabled  TRSumVariant=TrackingMode  SumFdbkVariant=Disabled  SumVariant=Sum_PID  TsampFilterVariant=InternalTs  TsampNgainVariant=Passthrough  TsampIntegralVariant=Disabled_SignalSpec  ExternalSaturationOutDataTypeStr=Inherit: Same as second input  DerivativeSourceVariant=ErrorSignal  PreIntVariant=InternalPreInt
  y : Outport
  wires:
  PID Controller2/1 -> y/1
  theta_track/1 -> PID Controller2/2
  e_h/1 -> PID Controller2/1

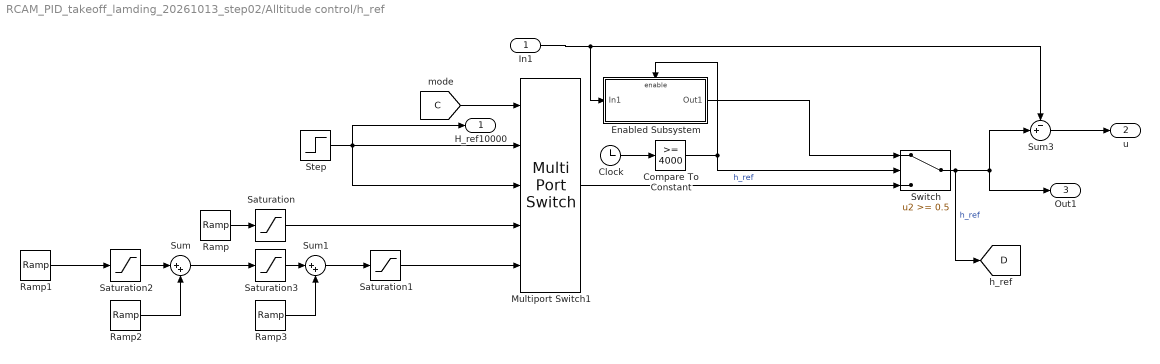
== system RCAM_PID_takeoff_lamding_20261013_step02/Alltitude control/h_ref ==
  In1 : Inport
  Clock : Clock
  Compare To Constant : simulink/Logic and Bit Operations/Compare To Constant  relop=>=  const=4000  OutDataTypeStr=boolean
  Enabled Subsystem : Subsystem  TreatAsAtomicUnit=on
  Multiport Switch1 : MultiPortSwitch  Inputs=4  SaturateOnIntegerOverflow=off  InputSameDT=off
  Ramp : simulink/Sources/Ramp  slope=-3  start=300  InitialOutput=10000*0.3048
  Ramp1 : simulink/Sources/Ramp  slope=-3  start=1500  InitialOutput=2000
  Ramp2 : simulink/Sources/Ramp  slope=-3  start=1900  InitialOutput=0
  Ramp3 : simulink/Sources/Ramp  slope=-1  start=3200  InitialOutput=0
  Saturation : Saturate  UpperLimit=10000*0.3048  LowerLimit=2000
  Saturation1 : Saturate  UpperLimit=inf  LowerLimit=50
  Saturation2 : Saturate  UpperLimit=inf  LowerLimit=1500
  Saturation3 : Saturate  UpperLimit=inf  LowerLimit=300
  Step : Step  Time=500  Before=3100  After=3100  SampleTime=0
  Sum : Sum  Inputs=|++
  Sum1 : Sum  Inputs=|++
  Sum3 : Sum  Inputs=-+|
  Switch : Switch  Threshold=0.5  SaturateOnIntegerOverflow=off  InputSameDT=off
  H_ref10000 : Outport
  u : Outport  Port=2
  Out1 : Outport  Port=3
  tag scope: D=global
  wires:
  Saturation1/1 -> Multiport Switch1/5
  Saturation/1 -> Multiport Switch1/4
  Step/1 -> H_ref10000/1, Multiport Switch1/3, Multiport Switch1/2
  Ramp/1 -> Saturation/1
  Ramp1/1 -> Saturation2/1
  Sum3/1 -> u/1
  In1/1 -> Sum3/1, Enabled Subsystem/1(In1)
  [C] -> Multiport Switch1/1
  Switch/1 -> [D], Sum3/2, Out1/1  "h_ref"
  Saturation2/1 -> Sum/1
  Sum/1 -> Saturation3/1
  Ramp2/1 -> Sum/2
  Saturation3/1 -> Sum1/1
  Sum1/1 -> Saturation1/1
  Ramp3/1 -> Sum1/2
  Clock/1 -> Compare To Constant/1
  Compare To Constant/1 -> Switch/2, Enabled Subsystem/Enable
  Multiport Switch1/1 -> Switch/3  "h_ref"
  Enabled Subsystem/1(Out1) -> Switch/1

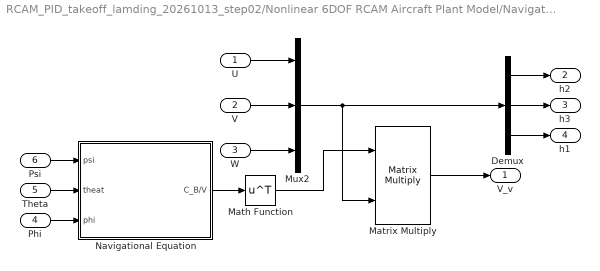
== system RCAM_PID_takeoff_lamding_20261013_step02/Nonlinear 6DOF RCAM Aircraft Plant Model/Navigational BLOCK ==
  U : Inport
  V : Inport  Port=2
  W : Inport  Port=3
  Phi : Inport  Port=4
  Theta : Inport  Port=5
  Psi : Inport  Port=6
  Demux : Demux  Outputs=3
  Math Function : Math  Operator=transpose
  Matrix Multiply : Product  Multiplication=Matrix(*)
  Mux2 : Mux  Inputs=3
  Navigational Equation : Subsystem
  V_v : Outport
  h2 : Outport  Port=2
  h3 : Outport  Port=3
  h1 : Outport  Port=4
  wires:
  V/1 -> Mux2/2
  Psi/1 -> Navigational Equation/1(psi)
  W/1 -> Mux2/3
  Navigational Equation/1(C_B/V) -> Math Function/1
  Matrix Multiply/1 -> V_v/1
  Theta/1 -> Navigational Equation/2(theat)
  U/1 -> Mux2/1
  Phi/1 -> Navigational Equation/3(phi)
  Math Function/1 -> Matrix Multiply/1
  Mux2/1 -> Matrix Multiply/2, Demux/1
  Demux/1 -> h2/1
  Demux/2 -> h3/1
  Demux/3 -> h1/1

== system RCAM_PID_takeoff_lamding_20261013_step02/Alltitude control/Subsystem/Triggered Subsystem ==
  In1 : Inport
  Trigger : TriggerPort  VariantControl=(inherit)
  Out1 : Outport  InitialOutput=9999
  wires:
  In1/1 -> Out1/1

== system RCAM_PID_takeoff_lamding_20261013_step02/Alltitude control/Subsystem/Triggered Subsystem1 ==
  In1 : Inport
  Trigger : TriggerPort  VariantControl=(inherit)
  Out1 : Outport  InitialOutput=9999
  wires:
  In1/1 -> Out1/1

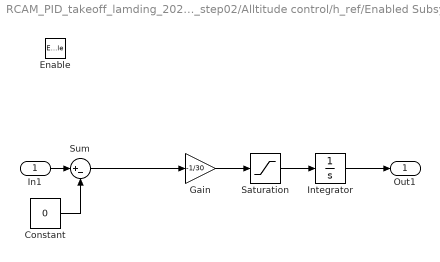
== system RCAM_PID_takeoff_lamding_20261013_step02/Alltitude control/h_ref/Enabled Subsystem ==
  In1 : Inport
  Enable : EnablePort  StatesWhenEnabling=reset
  Constant : Constant  Value=0
  Gain : Gain  Gain=-1/30
  Integrator : Integrator  InitialCondition=50  LimitOutput=on  LowerSaturationLimit=-0.5
  Saturation : Saturate  UpperLimit=-0.3  LowerLimit=-1
  Sum : Sum  Inputs=|+-
  Out1 : Outport
  wires:
  In1/1 -> Sum/1
  Sum/1 -> Gain/1
  Constant/1 -> Sum/2
  Gain/1 -> Saturation/1
  Saturation/1 -> Integrator/1
  Integrator/1 -> Out1/1
